simulink model "sschdlexMMCModel"  (R2026a)
settings: Solver=FixedStepDiscrete  StopTime=0.5
PostLoadFcn:
  | N = 5; % Number of Half-bridge Sub modules
  | Vdc = 640e3; % Input DC Voltage
InitFcn:
  | % Controller Parameters
  | m = 0.8; % Modulation Index of reference AC signals
  | f_out = 60; % Frequency of reference AC signals
  | Ts_CPU = 5e-5; % CPU sample time
  | 
  | % Plant Parameters
  | Ld = 30e-3; % Arm Inductance
  | Rd = 5; % Arm Resistance
  | Cm = 2e-3; % Capacitance
  | RL = 232.5; % Load Resistance
  | L = 50e-3; % Load Inductance
  | Ts_FPGA = 1e-6; % FPGA sample time
  | 
  | % PWM Generator Parameters
  | fsw = 1000; % Switching frequency
  | Tper = 1/(fsw); % Time period
  | Tdelay = 0:Tper/N:Tper*(N-1)/N; % Delay in the carrier signals
undefined symbols (not defined in the file or in its folder): DiscIntNeverNeededParam
libraries: fl_lib x30, nesl_utility x21, ee_lib x9
settings Model: DataTypeOverride=Off  Creator=The MathWorks, Inc.  LastModifiedBy=The MathWorks, Inc.
settings OptimizationCC: ConditionallyExecuteInputs=off  InheritOutputTypeSmallerThanSingle=on
settings DebuggingCC: ArtificialAlgebraicLoopMsg=error  SingleTaskRateTransMsg=error  ParameterPrecisionLossMsg=none
settings HardwareCC: ProdHWDeviceType=ASIC/FPGA->ASIC/FPGA  TargetBitPerLong=64.0  TargetBitPerPointer=64.0  TargetBitPerSizeT=64.0  TargetBitPerPtrDiffT=64.0  TargetLongLongMode=on  TargetIntDivRoundTo=Zero  TargetEndianess=LittleEndian  TargetWordSize=64.0  TargetHWDeviceType=Custom Processor->MATLAB Host Computer  ProdEqTarget=off
settings SimscapeCC: SimscapeNominalValues="[{\"value\":\"1\",\"unit\":\"A\"},{\"value\":\"1\",\"unit\":\"bar\"},{\"value\":\"1\",\"unit\":\"cm^2\"},{\"value\":\"1\",\"unit\":\"cm^3/s\"},{\"value\":\"1\",\"unit\":\"kJ/kg\"},{\"value\":\"1\",\"unit\":\"kW\"},{\"value\":\"1\",\"unit\":\"l\"},{\"value\":\"1\",\"unit\":\"N\"},{\"value\":\"1\",\"unit\":\"N*m\"},{\"value\":\"1\",\"unit\":\"V\"}]"  SimscapeLogType=none  SimscapeLogDataHistory=5000.0

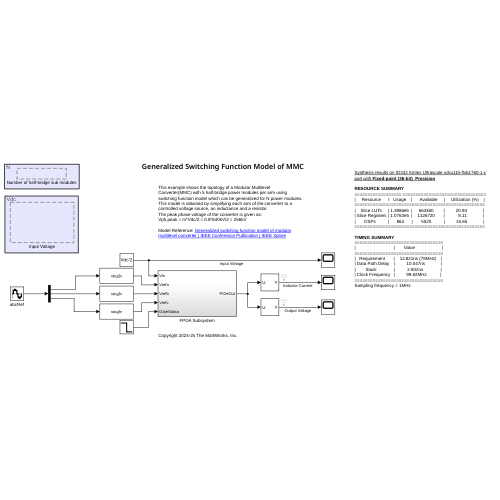
[thumbnail: Simulink's stored preview of the top-level diagram]
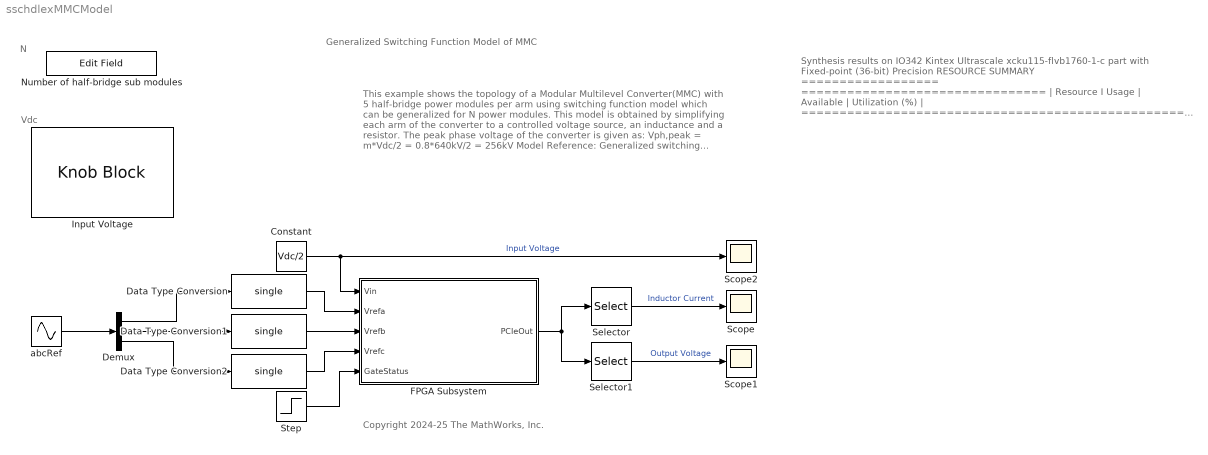
== system sschdlexMMCModel ==
  note: N
  note: Copyright 2024-25 The MathWorks, Inc.
  note: This example shows the topology of a Modular Multilevel Converter(MMC) with 5 half-bridge power modules per arm using switching function model which can be generalized for N power modules.
      | This model is obtained by simplifying each arm of the converter to a controlled voltage source, an inductance and a resistor.
      | The peak phase voltage of the converter is given as:
      | Vph,peak = m*Vdc/2 = 0.8*640kV/2 = 256kV
      |
      | Model Reference: Generalized switching function model of modular multilevel converter | IEEE Conference Publication | IEEE Xplore
  note: Synthesis results on IO342 Kintex Ultrascale xcku115-flvb1760-1-c part with Fixed-point (36-bit) Precision
      |
      | RESOURCE SUMMARY
      | ================== ================================
      | | Resource I Usage | Available | Utilization (%) |
      | ==================================================
      | | Slice LUTs | 1.3886e5 | 663360 | 20.93 |
      | | Slice Registers | 1.0763e5 | 1326720 | 8.11 |
      | | DSPs | 864 | 5520 | 15.65 |
      | ==================================================
      |
      | TIMING SUMMARY
      | ==================================
      | | | Value |
      | ==================================
      | | Requirement | 12.821ns (78MHz) |
      | | Data Path Delay | 10.047ns |
      | | Slack | 2.802ns |
      | | Clock Frequency | 99.82MHz |
      | ==================================
      | Sampling frequency = 1MHz
  note: Vdc
  note: Generalized Switching Function Model of MMC
  Constant : Constant  Value=Vdc/2  OutDataTypeStr=single  SampleTime=5e-5
  Data Type Conversion : DataTypeConversion  OutDataTypeStr=single  SaturateOnIntegerOverflow=off  RndMeth=Floor
  Data Type Conversion1 : DataTypeConversion  OutDataTypeStr=single  SaturateOnIntegerOverflow=off  RndMeth=Floor
  Data Type Conversion2 : DataTypeConversion  OutDataTypeStr=single  SaturateOnIntegerOverflow=off  RndMeth=Floor
  Demux : Demux  Outputs=3
  FPGA Subsystem : Subsystem
  Input Voltage : KnobBlock  LabelPosition=Hide  ScaleMin=2e5  ScaleMax=7e5  TickInterval=5e4
  Number of half-bridge sub modules : EditField  LabelPosition=Hide  ShowInitialText=on  Alignment=Center
  Scope : Scope
      settings: ActiveDisplayYMinimum=-1  ActiveDisplayYMaximum=1
  Scope1 : Scope
      settings: ActiveDisplayYMinimum=200918.97954337002  ActiveDisplayYMaximum=313521.80825799267  DataLoggingVariableName=ScopeData2
  Scope2 : Scope
      settings: ActiveDisplayYMinimum=220000  ActiveDisplayYMaximum=420000
  Selector : Selector  InputPortWidth=6  IndexOptions=Index vector (dialog)  Indices=[1:3]  OutputSizes=1
  Selector1 : Selector  InputPortWidth=6  IndexOptions=Index vector (dialog)  Indices=[4:6]  OutputSizes=1
  Step : Step  Time=0.25  InitialValue=1  FinalValue=0  SampleTime=5e-5
  abcRef : Sin  Amplitude=m  Frequency=2*pi*f_out  Phase=[0 -2*pi/3 2*pi/3]  SampleTime=Ts_CPU
  wires:
  Demux/1 -> Data Type Conversion/1
  Data Type Conversion1/1 -> FPGA Subsystem/3(Vrefb)
  Selector/1 -> Scope/1  "Inductor Current"
  Data Type Conversion2/1 -> FPGA Subsystem/4(Vrefc)
  Demux/3 -> Data Type Conversion2/1
  Demux/2 -> Data Type Conversion1/1
  FPGA Subsystem/1(PCIeOut) -> Selector1/1, Selector/1
  abcRef/1 -> Demux/1
  Selector1/1 -> Scope1/1  "Output Voltage"
  Constant/1 -> FPGA Subsystem/1(Vin), Scope2/1  "Input Voltage"
  Data Type Conversion/1 -> FPGA Subsystem/2(Vrefa)
  Step/1 -> FPGA Subsystem/5(GateStatus)

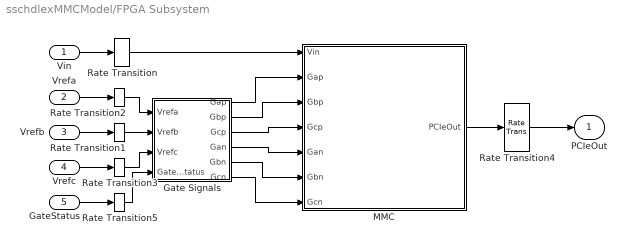
== system sschdlexMMCModel/FPGA Subsystem ==
  Vin : Inport
  Vrefa : Inport  Port=2
  Vrefb : Inport  Port=3
  Vrefc : Inport  Port=4
  GateStatus : Inport  Port=5
  Gate Signals : Subsystem
  MMC : Subsystem
  Rate Transition{,1..3,5} (5 alike) : RateTransition
  Rate Transition4 : RateTransition  OutPortSampleTime=Ts_CPU
  PCIeOut : Outport
  wires:
  Vrefc/1 -> Rate Transition3/1
  Vrefb/1 -> Rate Transition1/1
  Vrefa/1 -> Rate Transition2/1
  MMC/1(PCIeOut) -> Rate Transition4/1
  Vin/1 -> Rate Transition/1
  Rate Transition1/1 -> Gate Signals/2(Vrefb)
  Rate Transition2/1 -> Gate Signals/1(Vrefa)
  Rate Transition3/1 -> Gate Signals/3(Vrefc)
  Rate Transition4/1 -> PCIeOut/1
  Rate Transition/1 -> MMC/1(Vin)
  Gate Signals/1(Gap) -> MMC/2(Gap)
  Gate Signals/2(Gbp) -> MMC/3(Gbp)
  Gate Signals/3(Gcp) -> MMC/4(Gcp)
  Gate Signals/4(Gan) -> MMC/5(Gan)
  Gate Signals/5(Gbn) -> MMC/6(Gbn)
  Gate Signals/6(Gcn) -> MMC/7(Gcn)
  GateStatus/1 -> Rate Transition5/1
  Rate Transition5/1 -> Gate Signals/4(GateStatus)

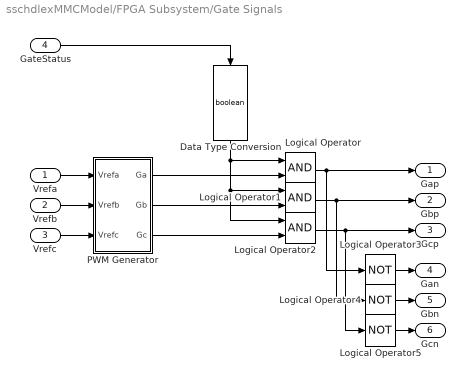
== system sschdlexMMCModel/FPGA Subsystem/Gate Signals ==
  Vrefa : Inport
  Vrefb : Inport  Port=2
  Vrefc : Inport  Port=3
  GateStatus : Inport  Port=4
  Data Type Conversion : DataTypeConversion  OutDataTypeStr=boolean  SaturateOnIntegerOverflow=off  RndMeth=Floor
  Logical Operator : Logic  AllPortsSameDT=off  OutDataTypeStr=boolean
  Logical Operator1 : Logic  AllPortsSameDT=off  OutDataTypeStr=boolean
  Logical Operator2 : Logic  AllPortsSameDT=off  OutDataTypeStr=boolean
  Logical Operator3 : Logic  Operator=NOT  AllPortsSameDT=off  OutDataTypeStr=boolean
  Logical Operator4 : Logic  Operator=NOT  AllPortsSameDT=off  OutDataTypeStr=boolean
  Logical Operator5 : Logic  Operator=NOT  AllPortsSameDT=off  OutDataTypeStr=boolean
  PWM Generator : Subsystem
  Gap : Outport
  Gbp : Outport  Port=2
  Gcp : Outport  Port=3
  Gan : Outport  Port=4
  Gbn : Outport  Port=5
  Gcn : Outport  Port=6
  wires:
  GateStatus/1 -> Data Type Conversion/1
  Logical Operator/1 -> Logical Operator3/1, Gap/1
  Data Type Conversion/1 -> Logical Operator2/1, Logical Operator1/1, Logical Operator/1
  Logical Operator2/1 -> Gcp/1, Logical Operator5/1
  Logical Operator1/1 -> Logical Operator4/1, Gbp/1
  Logical Operator3/1 -> Gan/1
  Logical Operator4/1 -> Gbn/1
  Logical Operator5/1 -> Gcn/1
  Vrefa/1 -> PWM Generator/1(Vrefa)
  Vrefb/1 -> PWM Generator/2(Vrefb)
  Vrefc/1 -> PWM Generator/3(Vrefc)
  PWM Generator/1(Ga) -> Logical Operator/2
  PWM Generator/2(Gb) -> Logical Operator1/2
  PWM Generator/3(Gc) -> Logical Operator2/2

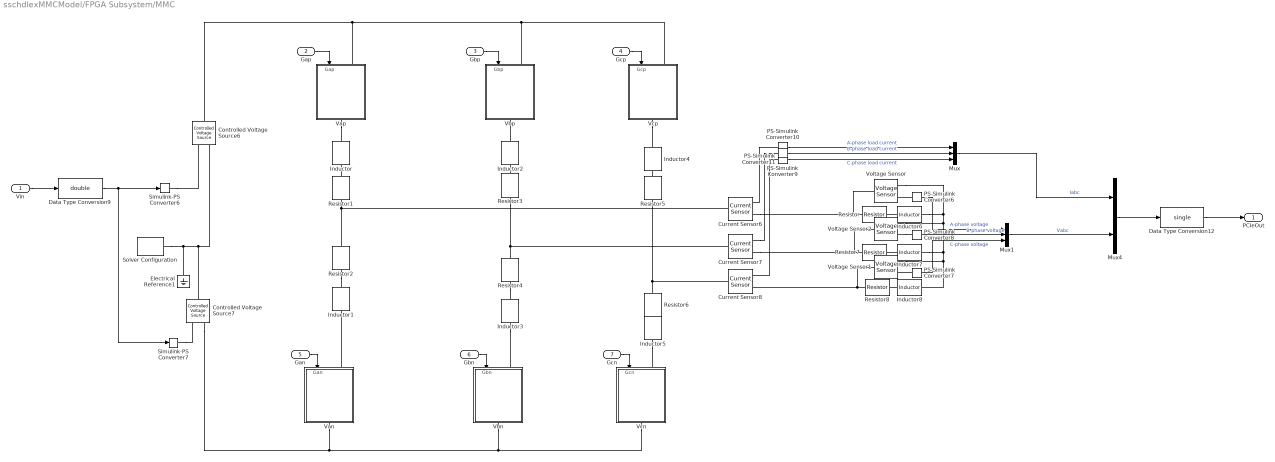
== system sschdlexMMCModel/FPGA Subsystem/MMC ==
  Vin : Inport
  Gap : Inport  Port=2
  Gbp : Inport  Port=3
  Gcp : Inport  Port=4
  Gan : Inport  Port=5
  Gbn : Inport  Port=6
  Gcn : Inport  Port=7
  Controlled Voltage Source6 : fl_lib/Electrical/Electrical Sources/Controlled Voltage Source
  Controlled Voltage Source7 : fl_lib/Electrical/Electrical Sources/Controlled Voltage Source
  Current Sensor6 : fl_lib/Electrical/Electrical Sensors/Current Sensor
  Current Sensor7 : fl_lib/Electrical/Electrical Sensors/Current Sensor
  Current Sensor8 : fl_lib/Electrical/Electrical Sensors/Current Sensor
  Data Type Conversion12 : DataTypeConversion  OutDataTypeStr=single  SaturateOnIntegerOverflow=off  RndMeth=Floor
  Data Type Conversion9 : DataTypeConversion  OutDataTypeStr=double  SaturateOnIntegerOverflow=off  RndMeth=Floor
  Electrical Reference1 : fl_lib/Electrical/Electrical Elements/Electrical Reference
  Inductor{,1..5} (6 alike) : ee_lib/Passive/Inductor  l=Ld H  enable_L_tol=ee.enum.toleranceApplication.none  L_tol=20  tol_distribution=ee.enum.toleranceDistribution.uniform  nSigma=4  r=0 Ohm  g=1e-9 1/Ohm  enable_operating_limits=ee.enum.enable.no  operating_limit_action=ee.enum.passive.reportOpLim.warn  max_working_current=1 A  power_rating=1 W  i_L_specify=off  i_L_priority=High  i_L=0 A  i_L_nominal_specify=off  i_L_nominal_value=1  i_L_nominal_unit=A
  Inductor6 : ee_lib/Passive/Inductor  l=L H  enable_L_tol=ee.enum.toleranceApplication.none  L_tol=20  tol_distribution=ee.enum.toleranceDistribution.uniform  nSigma=4  r=0 Ohm  g=1e-9 1/Ohm  enable_operating_limits=ee.enum.enable.no  operating_limit_action=ee.enum.passive.reportOpLim.warn  max_working_current=1 A  power_rating=1 W  i_L_specify=off  i_L_priority=High  i_L=0 A  i_L_nominal_specify=off  i_L_nominal_value=1  i_L_nominal_unit=A
  Inductor7 : ee_lib/Passive/Inductor  l=L H  enable_L_tol=ee.enum.toleranceApplication.none  L_tol=20  tol_distribution=ee.enum.toleranceDistribution.uniform  nSigma=4  r=0 Ohm  g=1e-9 1/Ohm  enable_operating_limits=ee.enum.enable.no  operating_limit_action=ee.enum.passive.reportOpLim.warn  max_working_current=1 A  power_rating=1 W  i_L_specify=off  i_L_priority=High  i_L=0 A  i_L_nominal_specify=off  i_L_nominal_value=1  i_L_nominal_unit=A
  Inductor8 : ee_lib/Passive/Inductor  l=L H  enable_L_tol=ee.enum.toleranceApplication.none  L_tol=20  tol_distribution=ee.enum.toleranceDistribution.uniform  nSigma=4  r=0 Ohm  g=1e-9 1/Ohm  enable_operating_limits=ee.enum.enable.no  operating_limit_action=ee.enum.passive.reportOpLim.warn  max_working_current=1 A  power_rating=1 W  i_L_specify=off  i_L_priority=High  i_L=0 A  i_L_nominal_specify=off  i_L_nominal_value=1  i_L_nominal_unit=A
  Mux : Mux  Inputs=3
  Mux1 : Mux  Inputs=3
  Mux4 : Mux  Inputs=2
  PS-Simulink Converter{6..11} (6 alike) : nesl_utility/PS-Simulink Converter  PhysicalDomain=network_engine_domain  SubClassName=ps_output  LeftPortType=input  RightPortType=output  PseudoPeriodic=off  Frequencies=[]  VectorFormat=inherit  Unit=inherit  AffineConversion=off
  Resistor : fl_lib/Electrical/Electrical Elements/Resistor  R=RL Ohm  i_specify=off  i_priority=None  i=0 A  i_nominal_specify=off  i_nominal_value=1  i_nominal_unit=A  v_specify=off  v_priority=None  v=0 V  v_nominal_specify=off  v_nominal_value=1  v_nominal_unit=V
  Resistor{1..6} (6 alike) : fl_lib/Electrical/Electrical Elements/Resistor  R=Rd Ohm  i_specify=off  i_priority=None  i=0 A  i_nominal_specify=off  i_nominal_value=1  i_nominal_unit=A  v_specify=off  v_priority=None  v=0 V  v_nominal_specify=off  v_nominal_value=1  v_nominal_unit=V
  Resistor7 : fl_lib/Electrical/Electrical Elements/Resistor  R=RL Ohm  i_specify=off  i_priority=None  i=0 A  i_nominal_specify=off  i_nominal_value=1  i_nominal_unit=A  v_specify=off  v_priority=None  v=0 V  v_nominal_specify=off  v_nominal_value=1  v_nominal_unit=V
  Resistor8 : fl_lib/Electrical/Electrical Elements/Resistor  R=RL Ohm  i_specify=off  i_priority=None  i=0 A  i_nominal_specify=off  i_nominal_value=1  i_nominal_unit=A  v_specify=off  v_priority=None  v=0 V  v_nominal_specify=off  v_nominal_value=1  v_nominal_unit=V
  Simulink-PS Converter6 : nesl_utility/Simulink-PS Converter  PhysicalDomain=network_engine_domain  SubClassName=ps_input  LeftPortType=input  RightPortType=output  PseudoPeriodic=off  Frequencies=[]  NoiseDistribution=none  NoiseParameters=[]  Unit=1  AffineConversion=off  FilteringAndDerivatives=provide  SimscapeFilterOrder=1  InputFilterTimeConstant=0.001  UdotUserProvided=0
  Simulink-PS Converter7 : nesl_utility/Simulink-PS Converter  PhysicalDomain=network_engine_domain  SubClassName=ps_input  LeftPortType=input  RightPortType=output  PseudoPeriodic=off  Frequencies=[]  NoiseDistribution=none  NoiseParameters=[]  Unit=1  AffineConversion=off  FilteringAndDerivatives=provide  SimscapeFilterOrder=1  InputFilterTimeConstant=0.001  UdotUserProvided=0
  Solver Configuration : nesl_utility/Solver Configuration  PhysicalDomain=network_engine_domain  SubClassName=solver  LeftPortType=input  RightPortType=generic  Tones=[]  Harmonics=[]  SimulateNoise=off  Profile=off  UseLocalSampling=off  EnableSwitchedLinearOptims=on  FrequencyDomain=off  UseCCode=off  RelTol=0.001  AbsTol=0.001  MinStep=1e-09  ToWorkspace=off  RevertToSquareIcSolve=off  NumHomotopyIterations=100  PhasorMode=off  PhasorModeNumHarmonics=1  ConsistencySolver=NEWTON_XTOL_AFTER_FTOL  CanonicalOrdering=UNORDERED  OptimizeIntermediates=UNOPTIMIZED  IndexReductionMethod=DerivativeReplacement  DoDC=off  ResidualTolerance=1e-09  ConsistencyTolSource=GLOBAL  ConsistencyAbsTol=0.001  ConsistencyRelTol=0.001  ConsistencyTolFactor=0.001  UseLocalSolver=on  LocalSolverChoice=NE_BACKWARD_EULER_ADVANCER  ResolveIndetEquations=off  FunctionEvalNumThread=1  LocalSolverSampleTime=Ts_FPGA  DoFixedCost=off  MaxNonlinIter=3  MaxModeIter=2  ComputeImpulses=off  ImpulseIterations=2  LinearAlgebra=auto  LinearAlgebraNumThread=0  EquationFormulation=NE_TIME_EF  DelaysMemoryBudget=1024  AutomaticFiltering=on  FilteringTimeConstant=0.001  PartitionStorageMethod=AS_NEEDED  PartitionMemoryBudget=1024  PartitionMethod=ROBUST  MultibodyUseLocalSolver=off  MultibodyLocalSolverChoice=ODE1  MultibodyLocalSolverSampleTime=0.001
  Van : Subsystem
  Vap : Subsystem
  Vbn : Subsystem
  Vbp : Subsystem
  Vcn : Subsystem
  Vcp : Subsystem
  Voltage Sensor : fl_lib/Electrical/Electrical Sensors/Voltage Sensor
  Voltage Sensor1 : fl_lib/Electrical/Electrical Sensors/Voltage Sensor
  Voltage Sensor2 : fl_lib/Electrical/Electrical Sensors/Voltage Sensor
  PCIeOut : Outport
  wires:
  Data Type Conversion12/1 -> PCIeOut/1
  Gcn/1 -> Vcn/1(Gcn)
  Gbn/1 -> Vbn/1(Gbn)
  Gcp/1 -> Vcp/1(Gcp)
  Gbp/1 -> Vbp/1(Gbp)
  Gan/1 -> Van/1(Gan)
  Gap/1 -> Vap/1(Gap)
  Data Type Conversion9/1 -> Simulink-PS Converter7/1, Simulink-PS Converter6/1
  Vin/1 -> Data Type Conversion9/1
  Mux4/1 -> Data Type Conversion12/1
  Mux1/1 -> Mux4/2  "Vabc"
  Mux/1 -> Mux4/1  "Iabc"
  PS-Simulink Converter10/1 -> Mux/1  "A-phase load current"
  PS-Simulink Converter6/1 -> Mux1/1  "A-phase voltage"
  PS-Simulink Converter8/1 -> Mux1/2  "B-phase voltage"
  PS-Simulink Converter7/1 -> Mux1/3  "C-phase voltage"
  PS-Simulink Converter11/1 -> Mux/3  "C-phase load current"
  PS-Simulink Converter9/1 -> Mux/2  "B-phase load current"
  connections:
  Inductor5/RConn1 -- Vcn/LConn1
  Inductor3/RConn1 -- Vbn/LConn1
  Current Sensor6/LConn1 -- Resistor2/LConn1 -- Resistor1/RConn1
  Vap/RConn1 -- Inductor/LConn1
  Inductor2/LConn1 -- Vbp/RConn1
  Resistor1/LConn1 -- Inductor/RConn1
  Controlled Voltage Source6/LConn1 -- Vcp/LConn1 -- Vbp/LConn1 -- Vap/LConn1
  Van/LConn1 -- Inductor1/RConn1
  Simulink-PS Converter7/RConn1 -- Controlled Voltage Source7/RConn1
  Simulink-PS Converter6/RConn1 -- Controlled Voltage Source6/RConn1
  Voltage Sensor2/RConn1 -- PS-Simulink Converter8/LConn1
  Solver Configuration/RConn1 -- Electrical Reference1/LConn1 -- Controlled Voltage Source6/RConn2 -- Controlled Voltage Source7/LConn1
  Inductor7/LConn1 -- Resistor7/RConn1
  Resistor4/RConn1 -- Inductor3/LConn1
  Vcp/RConn1 -- Inductor4/LConn1
  Inductor8/LConn1 -- Resistor8/RConn1
  PS-Simulink Converter10/LConn1 -- Current Sensor6/RConn1
  Resistor2/RConn1 -- Inductor1/LConn1
  Resistor6/RConn1 -- Inductor5/LConn1
  Resistor3/LConn1 -- Inductor2/RConn1
  Inductor6/LConn1 -- Resistor/RConn1
  PS-Simulink Converter11/LConn1 -- Current Sensor8/RConn1
  Voltage Sensor2/LConn1 -- Current Sensor7/RConn2 -- Resistor7/LConn1
  Controlled Voltage Source7/RConn2 -- Vcn/RConn1 -- Vbn/RConn1 -- Van/RConn1
  PS-Simulink Converter7/LConn1 -- Voltage Sensor1/RConn1
  Current Sensor7/RConn1 -- PS-Simulink Converter9/LConn1
  Current Sensor8/LConn1 -- Resistor5/RConn1 -- Resistor6/LConn1
  Inductor6/RConn1 -- Voltage Sensor/RConn2 -- Inductor8/RConn1 -- Voltage Sensor1/RConn2 -- Inductor7/RConn1 -- Voltage Sensor2/RConn2
  Resistor5/LConn1 -- Inductor4/RConn1
  PS-Simulink Converter6/LConn1 -- Voltage Sensor/RConn1
  Current Sensor7/LConn1 -- Resistor3/RConn1 -- Resistor4/LConn1
  Voltage Sensor1/LConn1 -- Current Sensor8/RConn2 -- Resistor8/LConn1
  Resistor/LConn1 -- Current Sensor6/RConn2 -- Voltage Sensor/LConn1

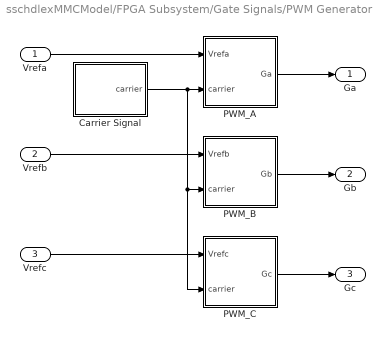
== system sschdlexMMCModel/FPGA Subsystem/Gate Signals/PWM Generator ==
  Vrefa : Inport
  Vrefb : Inport  Port=2
  Vrefc : Inport  Port=3
  Carrier Signal : Subsystem
  PWM_A : Subsystem  mask{N=N}
      mask prompts: N "Number of half-bridge sub modules"
      mask init:
      | PwmOutSelect = zeros(1,2*N);
      | PwmOutSelect(1:2:end) = 1:N;
      | PwmOutSelect(2:2:end) = N+1:2*N;
      mask DialogControl DescTextVar Prompt: PWM (a-phase)
  PWM_B : Subsystem  mask{N=N}
      mask prompts: N "Number of half-bridge sub modules"
      mask init:
      | PwmOutSelect = zeros(1,2*N);
      | PwmOutSelect(1:2:end) = 1:N;
      | PwmOutSelect(2:2:end) = N+1:2*N;
      mask DialogControl DescTextVar Prompt: PWM (b-phase)
  PWM_C : Subsystem  mask{N=N}
      mask prompts: N "Number of half-bridge sub modules"
      mask init:
      | PwmOutSelect = zeros(1,2*N);
      | PwmOutSelect(1:2:end) = 1:N;
      | PwmOutSelect(2:2:end) = N+1:2*N;
      mask DialogControl DescTextVar Prompt: PWM (c-phase)
  Ga : Outport
  Gb : Outport  Port=2
  Gc : Outport  Port=3
  wires:
  Vrefc/1 -> PWM_C/1(Vrefc)
  Vrefb/1 -> PWM_B/1(Vrefb)
  PWM_C/1(Gc) -> Gc/1
  Carrier Signal/1(carrier) -> PWM_C/2(carrier), PWM_B/2(carrier), PWM_A/2(carrier)
  Vrefa/1 -> PWM_A/1(Vrefa)
  PWM_B/1(Gb) -> Gb/1
  PWM_A/1(Ga) -> Ga/1

== system sschdlexMMCModel/FPGA Subsystem/MMC/Van ==
  Gan : Inport
  Controlled Voltage Source : fl_lib/Electrical/Electrical Sources/Controlled Voltage Source
  Current Sensor : fl_lib/Electrical/Electrical Sensors/Current Sensor
  Data Type Conversion : DataTypeConversion  OutDataTypeStr=double  SaturateOnIntegerOverflow=off  RndMeth=Floor
  Equivalent Voltage : Subsystem
  PS-Simulink Converter : nesl_utility/PS-Simulink Converter  PhysicalDomain=network_engine_domain  SubClassName=ps_output  LeftPortType=input  RightPortType=output  PseudoPeriodic=off  Frequencies=[]  VectorFormat=inherit  Unit=inherit  AffineConversion=off
  Simulink-PS Converter : nesl_utility/Simulink-PS Converter  PhysicalDomain=network_engine_domain  SubClassName=ps_input  LeftPortType=input  RightPortType=output  PseudoPeriodic=off  Frequencies=[]  NoiseDistribution=none  NoiseParameters=[]  Unit=1  AffineConversion=off  FilteringAndDerivatives=provide  SimscapeFilterOrder=1  InputFilterTimeConstant=0.001  UdotUserProvided=0
  + : PMIOPort  Side=Left
  - : PMIOPort  Port=2  Side=Right
  wires:
  Gan/1 -> Equivalent Voltage/1(Gan)
  Equivalent Voltage/1(van) -> Data Type Conversion/1
  PS-Simulink Converter/1 -> Equivalent Voltage/2(ian)
  Data Type Conversion/1 -> Simulink-PS Converter/1
  connections:
  +/RConn1 -- Controlled Voltage Source/LConn1
  Current Sensor/LConn1 -- Controlled Voltage Source/RConn2
  Current Sensor/RConn1 -- PS-Simulink Converter/LConn1
  -/RConn1 -- Current Sensor/RConn2
  Simulink-PS Converter/RConn1 -- Controlled Voltage Source/RConn1

== system sschdlexMMCModel/FPGA Subsystem/MMC/Vap ==
  Gap : Inport
  Controlled Voltage Source : fl_lib/Electrical/Electrical Sources/Controlled Voltage Source
  Current Sensor : fl_lib/Electrical/Electrical Sensors/Current Sensor
  Data Type Conversion : DataTypeConversion  OutDataTypeStr=double  SaturateOnIntegerOverflow=off  RndMeth=Floor
  Equivalent Voltage : Subsystem
  PS-Simulink Converter : nesl_utility/PS-Simulink Converter  PhysicalDomain=network_engine_domain  SubClassName=ps_output  LeftPortType=input  RightPortType=output  PseudoPeriodic=off  Frequencies=[]  VectorFormat=inherit  Unit=inherit  AffineConversion=off
  Simulink-PS Converter : nesl_utility/Simulink-PS Converter  PhysicalDomain=network_engine_domain  SubClassName=ps_input  LeftPortType=input  RightPortType=output  PseudoPeriodic=off  Frequencies=[]  NoiseDistribution=none  NoiseParameters=[]  Unit=1  AffineConversion=off  FilteringAndDerivatives=provide  SimscapeFilterOrder=1  InputFilterTimeConstant=0.001  UdotUserProvided=0
  + : PMIOPort  Side=Left
  - : PMIOPort  Port=2  Side=Right
  wires:
  Data Type Conversion/1 -> Simulink-PS Converter/1
  PS-Simulink Converter/1 -> Equivalent Voltage/2(iap)
  Equivalent Voltage/1(vap) -> Data Type Conversion/1
  Gap/1 -> Equivalent Voltage/1(Gap)
  connections:
  Simulink-PS Converter/RConn1 -- Controlled Voltage Source/RConn1
  -/RConn1 -- Current Sensor/RConn2
  Current Sensor/RConn1 -- PS-Simulink Converter/LConn1
  Current Sensor/LConn1 -- Controlled Voltage Source/RConn2
  +/RConn1 -- Controlled Voltage Source/LConn1

== system sschdlexMMCModel/FPGA Subsystem/MMC/Vbn ==
  Gbn : Inport
  Controlled Voltage Source : fl_lib/Electrical/Electrical Sources/Controlled Voltage Source
  Current Sensor : fl_lib/Electrical/Electrical Sensors/Current Sensor
  Data Type Conversion : DataTypeConversion  OutDataTypeStr=double  SaturateOnIntegerOverflow=off  RndMeth=Floor
  Equivalent Voltage : Subsystem
  PS-Simulink Converter : nesl_utility/PS-Simulink Converter  PhysicalDomain=network_engine_domain  SubClassName=ps_output  LeftPortType=input  RightPortType=output  PseudoPeriodic=off  Frequencies=[]  VectorFormat=inherit  Unit=inherit  AffineConversion=off
  Simulink-PS Converter : nesl_utility/Simulink-PS Converter  PhysicalDomain=network_engine_domain  SubClassName=ps_input  LeftPortType=input  RightPortType=output  PseudoPeriodic=off  Frequencies=[]  NoiseDistribution=none  NoiseParameters=[]  Unit=1  AffineConversion=off  FilteringAndDerivatives=provide  SimscapeFilterOrder=1  InputFilterTimeConstant=0.001  UdotUserProvided=0
  + : PMIOPort  Side=Left
  - : PMIOPort  Port=2  Side=Right
  wires:
  Data Type Conversion/1 -> Simulink-PS Converter/1
  PS-Simulink Converter/1 -> Equivalent Voltage/2(ibn)
  Equivalent Voltage/1(vbn) -> Data Type Conversion/1
  Gbn/1 -> Equivalent Voltage/1(Gbn)
  connections:
  Simulink-PS Converter/RConn1 -- Controlled Voltage Source/RConn1
  -/RConn1 -- Current Sensor/RConn2
  Current Sensor/RConn1 -- PS-Simulink Converter/LConn1
  Current Sensor/LConn1 -- Controlled Voltage Source/RConn2
  +/RConn1 -- Controlled Voltage Source/LConn1

== system sschdlexMMCModel/FPGA Subsystem/MMC/Vbp ==
  Gbp : Inport
  Controlled Voltage Source : fl_lib/Electrical/Electrical Sources/Controlled Voltage Source
  Current Sensor : fl_lib/Electrical/Electrical Sensors/Current Sensor
  Data Type Conversion : DataTypeConversion  OutDataTypeStr=double  SaturateOnIntegerOverflow=off  RndMeth=Floor
  Equivalent Voltage : Subsystem
  PS-Simulink Converter : nesl_utility/PS-Simulink Converter  PhysicalDomain=network_engine_domain  SubClassName=ps_output  LeftPortType=input  RightPortType=output  PseudoPeriodic=off  Frequencies=[]  VectorFormat=inherit  Unit=inherit  AffineConversion=off
  Simulink-PS Converter : nesl_utility/Simulink-PS Converter  PhysicalDomain=network_engine_domain  SubClassName=ps_input  LeftPortType=input  RightPortType=output  PseudoPeriodic=off  Frequencies=[]  NoiseDistribution=none  NoiseParameters=[]  Unit=1  AffineConversion=off  FilteringAndDerivatives=provide  SimscapeFilterOrder=1  InputFilterTimeConstant=0.001  UdotUserProvided=0
  + : PMIOPort  Side=Left
  - : PMIOPort  Port=2  Side=Right
  wires:
  Gbp/1 -> Equivalent Voltage/1(Gbp)
  Equivalent Voltage/1(vbp) -> Data Type Conversion/1
  PS-Simulink Converter/1 -> Equivalent Voltage/2(ibp)
  Data Type Conversion/1 -> Simulink-PS Converter/1
  connections:
  +/RConn1 -- Controlled Voltage Source/LConn1
  Current Sensor/LConn1 -- Controlled Voltage Source/RConn2
  Current Sensor/RConn1 -- PS-Simulink Converter/LConn1
  -/RConn1 -- Current Sensor/RConn2
  Simulink-PS Converter/RConn1 -- Controlled Voltage Source/RConn1

== system sschdlexMMCModel/FPGA Subsystem/MMC/Vcn ==
  Gcn : Inport
  Controlled Voltage Source : fl_lib/Electrical/Electrical Sources/Controlled Voltage Source
  Current Sensor : fl_lib/Electrical/Electrical Sensors/Current Sensor
  Data Type Conversion : DataTypeConversion  OutDataTypeStr=double  SaturateOnIntegerOverflow=off  RndMeth=Floor
  Equivalent Voltage : Subsystem
  PS-Simulink Converter : nesl_utility/PS-Simulink Converter  PhysicalDomain=network_engine_domain  SubClassName=ps_output  LeftPortType=input  RightPortType=output  PseudoPeriodic=off  Frequencies=[]  VectorFormat=inherit  Unit=inherit  AffineConversion=off
  Simulink-PS Converter : nesl_utility/Simulink-PS Converter  PhysicalDomain=network_engine_domain  SubClassName=ps_input  LeftPortType=input  RightPortType=output  PseudoPeriodic=off  Frequencies=[]  NoiseDistribution=none  NoiseParameters=[]  Unit=1  AffineConversion=off  FilteringAndDerivatives=provide  SimscapeFilterOrder=1  InputFilterTimeConstant=0.001  UdotUserProvided=0
  + : PMIOPort  Side=Left
  - : PMIOPort  Port=2  Side=Right
  wires:
  Gcn/1 -> Equivalent Voltage/1(Gcn)
  Equivalent Voltage/1(vcn) -> Data Type Conversion/1
  PS-Simulink Converter/1 -> Equivalent Voltage/2(icn)
  Data Type Conversion/1 -> Simulink-PS Converter/1
  connections:
  +/RConn1 -- Controlled Voltage Source/LConn1
  Current Sensor/LConn1 -- Controlled Voltage Source/RConn2
  Current Sensor/RConn1 -- PS-Simulink Converter/LConn1
  -/RConn1 -- Current Sensor/RConn2
  Simulink-PS Converter/RConn1 -- Controlled Voltage Source/RConn1

== system sschdlexMMCModel/FPGA Subsystem/MMC/Vcp ==
  Gcp : Inport
  Controlled Voltage Source : fl_lib/Electrical/Electrical Sources/Controlled Voltage Source
  Current Sensor : fl_lib/Electrical/Electrical Sensors/Current Sensor
  Data Type Conversion : DataTypeConversion  OutDataTypeStr=double  SaturateOnIntegerOverflow=off  RndMeth=Floor
  Equivalent Voltage : Subsystem
  PS-Simulink Converter : nesl_utility/PS-Simulink Converter  PhysicalDomain=network_engine_domain  SubClassName=ps_output  LeftPortType=input  RightPortType=output  PseudoPeriodic=off  Frequencies=[]  VectorFormat=inherit  Unit=inherit  AffineConversion=off
  Simulink-PS Converter : nesl_utility/Simulink-PS Converter  PhysicalDomain=network_engine_domain  SubClassName=ps_input  LeftPortType=input  RightPortType=output  PseudoPeriodic=off  Frequencies=[]  NoiseDistribution=none  NoiseParameters=[]  Unit=1  AffineConversion=off  FilteringAndDerivatives=provide  SimscapeFilterOrder=1  InputFilterTimeConstant=0.001  UdotUserProvided=0
  + : PMIOPort  Side=Left
  - : PMIOPort  Port=2  Side=Right
  wires:
  Data Type Conversion/1 -> Simulink-PS Converter/1
  PS-Simulink Converter/1 -> Equivalent Voltage/2(icp)
  Equivalent Voltage/1(vcp) -> Data Type Conversion/1
  Gcp/1 -> Equivalent Voltage/1(Gcp)
  connections:
  Simulink-PS Converter/RConn1 -- Controlled Voltage Source/RConn1
  -/RConn1 -- Current Sensor/RConn2
  Current Sensor/RConn1 -- PS-Simulink Converter/LConn1
  Current Sensor/LConn1 -- Controlled Voltage Source/RConn2
  +/RConn1 -- Controlled Voltage Source/LConn1

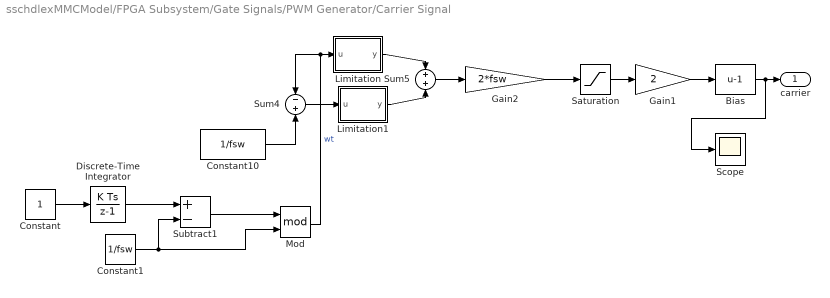
== system sschdlexMMCModel/FPGA Subsystem/Gate Signals/PWM Generator/Carrier Signal ==
  Bias : Bias  Bias=-1  SaturateOnIntegerOverflow=off
  Constant : Constant  OutDataTypeStr=single  SampleTime=-1
  Constant1 : Constant  Value=1/fsw  OutDataTypeStr=single  SampleTime=-1
  Constant10 : Constant  Value=1/fsw  OutDataTypeStr=single  SampleTime=-1
  Discrete-Time Integrator : DiscreteIntegrator  InitialCondition=Tdelay  SampleTime=-1  ICPrevOutput=DiscIntNeverNeededParam  ICPrevScaledInput=DiscIntNeverNeededParam
  Gain1 : Gain  Gain=2
  Gain2 : Gain  Gain=2*fsw
  Limitation : Subsystem
  Limitation1 : Subsystem
  Mod : Math  Operator=mod
  Saturation : Saturate  UpperLimit=1  LowerLimit=0
  Scope : Scope
      settings: ActiveDisplayYMinimum=-1.2499998658895493  ActiveDisplayYMaximum=1.2499987930059433  DataLoggingVariableName=ScopeData3
  Subtract1 : Sum  Inputs=+-
  Sum4 : Sum  Inputs=-+
  Sum5 : Sum
  carrier : Outport
  wires:
  Gain2/1 -> Saturation/1
  Saturation/1 -> Gain1/1
  Limitation/1(y) -> Sum5/1
  Subtract1/1 -> Mod/1
  Constant10/1 -> Sum4/2
  Mod/1 -> Limitation/1(u), Sum4/1  "wt"
  Constant1/1 -> Mod/2, Subtract1/2
  Sum5/1 -> Gain2/1
  Constant/1 -> Discrete-Time Integrator/1
  Gain1/1 -> Bias/1
  Limitation1/1(y) -> Sum5/2
  Discrete-Time Integrator/1 -> Subtract1/1
  Sum4/1 -> Limitation1/1(u)
  Bias/1 -> Scope/1, carrier/1

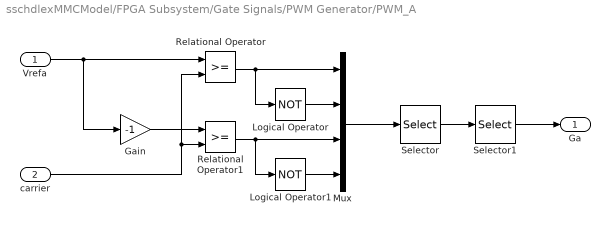
== system sschdlexMMCModel/FPGA Subsystem/Gate Signals/PWM Generator/PWM_A ==
  Vrefa : Inport
  carrier : Inport  Port=2
  Gain : Gain  Gain=-1
  Logical Operator : Logic  Operator=NOT  AllPortsSameDT=off  OutDataTypeStr=boolean
  Logical Operator1 : Logic  Operator=NOT  AllPortsSameDT=off  OutDataTypeStr=boolean
  Mux : Mux
  Relational Operator : RelationalOperator  OutDataTypeStr=boolean  RndMeth=Simplest  InputSameDT=off
  Relational Operator1 : RelationalOperator  OutDataTypeStr=boolean  RndMeth=Simplest  InputSameDT=off
  Selector : Selector  InputPortWidth=4*N  IndexOptions=Index vector (dialog)  Indices=PwmOutSelect  OutputSizes=1
  Selector1 : Selector  InputPortWidth=2*N  IndexOptions=Index vector (dialog)  Indices=[1:2:2*N]  OutputSizes=1
  Ga : Outport
  wires:
  Relational Operator1/1 -> Logical Operator1/1, Mux/3
  carrier/1 -> Relational Operator1/2, Relational Operator/2
  Vrefa/1 -> Gain/1, Relational Operator/1
  Mux/1 -> Selector/1
  Logical Operator/1 -> Mux/2
  Logical Operator1/1 -> Mux/4
  Selector/1 -> Selector1/1
  Relational Operator/1 -> Logical Operator/1, Mux/1
  Selector1/1 -> Ga/1
  Gain/1 -> Relational Operator1/1

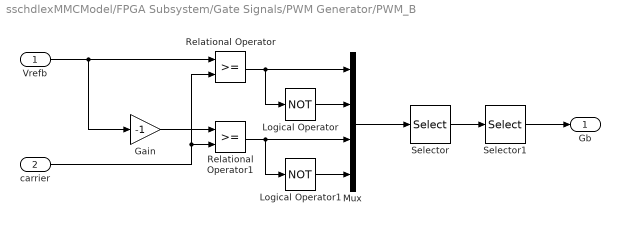
== system sschdlexMMCModel/FPGA Subsystem/Gate Signals/PWM Generator/PWM_B ==
  Vrefb : Inport
  carrier : Inport  Port=2
  Gain : Gain  Gain=-1
  Logical Operator : Logic  Operator=NOT  AllPortsSameDT=off  OutDataTypeStr=boolean
  Logical Operator1 : Logic  Operator=NOT  AllPortsSameDT=off  OutDataTypeStr=boolean
  Mux : Mux
  Relational Operator : RelationalOperator  OutDataTypeStr=boolean  RndMeth=Simplest  InputSameDT=off
  Relational Operator1 : RelationalOperator  OutDataTypeStr=boolean  RndMeth=Simplest  InputSameDT=off
  Selector : Selector  InputPortWidth=4*N  IndexOptions=Index vector (dialog)  Indices=PwmOutSelect  OutputSizes=1
  Selector1 : Selector  InputPortWidth=2*N  IndexOptions=Index vector (dialog)  Indices=[1:2:2*N]  OutputSizes=1
  Gb : Outport
  wires:
  Gain/1 -> Relational Operator1/1
  Selector1/1 -> Gb/1
  Relational Operator/1 -> Mux/1, Logical Operator/1
  Selector/1 -> Selector1/1
  Logical Operator1/1 -> Mux/4
  Logical Operator/1 -> Mux/2
  Mux/1 -> Selector/1
  Vrefb/1 -> Gain/1, Relational Operator/1
  carrier/1 -> Relational Operator/2, Relational Operator1/2
  Relational Operator1/1 -> Mux/3, Logical Operator1/1

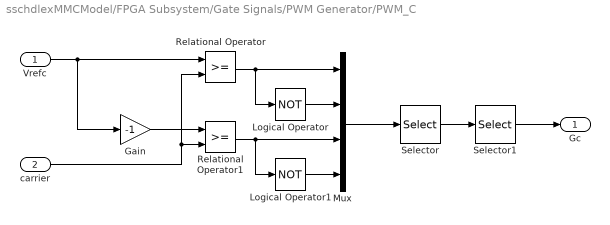
== system sschdlexMMCModel/FPGA Subsystem/Gate Signals/PWM Generator/PWM_C ==
  Vrefc : Inport
  carrier : Inport  Port=2
  Gain : Gain  Gain=-1
  Logical Operator : Logic  Operator=NOT  AllPortsSameDT=off  OutDataTypeStr=boolean
  Logical Operator1 : Logic  Operator=NOT  AllPortsSameDT=off  OutDataTypeStr=boolean
  Mux : Mux
  Relational Operator : RelationalOperator  OutDataTypeStr=boolean  RndMeth=Simplest  InputSameDT=off
  Relational Operator1 : RelationalOperator  OutDataTypeStr=boolean  RndMeth=Simplest  InputSameDT=off
  Selector : Selector  InputPortWidth=4*N  IndexOptions=Index vector (dialog)  Indices=PwmOutSelect  OutputSizes=1
  Selector1 : Selector  InputPortWidth=2*N  IndexOptions=Index vector (dialog)  Indices=[1:2:2*N]  OutputSizes=1
  Gc : Outport
  wires:
  Relational Operator1/1 -> Logical Operator1/1, Mux/3
  carrier/1 -> Relational Operator1/2, Relational Operator/2
  Vrefc/1 -> Gain/1, Relational Operator/1
  Mux/1 -> Selector/1
  Logical Operator/1 -> Mux/2
  Logical Operator1/1 -> Mux/4
  Selector/1 -> Selector1/1
  Relational Operator/1 -> Logical Operator/1, Mux/1
  Selector1/1 -> Gc/1
  Gain/1 -> Relational Operator1/1

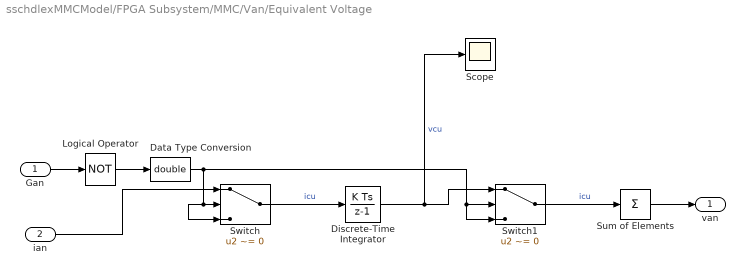
== system sschdlexMMCModel/FPGA Subsystem/MMC/Van/Equivalent Voltage ==
  Gan : Inport
  ian : Inport  Port=2
  Data Type Conversion : DataTypeConversion  OutDataTypeStr=double  SaturateOnIntegerOverflow=off  RndMeth=Floor
  Discrete-Time Integrator : DiscreteIntegrator  gainval=1/Cm  SampleTime=-1  ICPrevOutput=DiscIntNeverNeededParam  ICPrevScaledInput=DiscIntNeverNeededParam
  Logical Operator : Logic  Operator=NOT  AllPortsSameDT=off  OutDataTypeStr=boolean
  Scope : Scope
      settings: ActiveDisplayYMinimum=8640.12229  ActiveDisplayYMaximum=11210.56131  DataLoggingVariableName=ScopeData4
  Sum of Elements : Sum  Inputs=+
  Switch : Switch  Criteria=u2 ~= 0  SaturateOnIntegerOverflow=off  InputSameDT=off
  Switch1 : Switch  Criteria=u2 ~= 0  SaturateOnIntegerOverflow=off  InputSameDT=off
  van : Outport
  wires:
  Logical Operator/1 -> Data Type Conversion/1
  Switch1/1 -> Sum of Elements/1  "icu"
  ian/1 -> Switch/1
  Gan/1 -> Logical Operator/1
  Sum of Elements/1 -> van/1
  Switch/1 -> Discrete-Time Integrator/1  "icu"
  Discrete-Time Integrator/1 -> Switch1/1, Scope/1  "vcu"
  Data Type Conversion/1 -> Switch/2, Switch/3, Switch1/2, Switch1/3

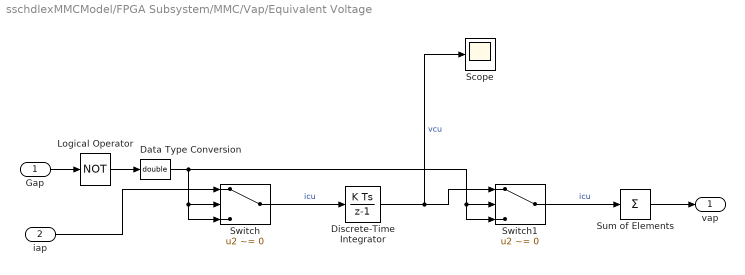
== system sschdlexMMCModel/FPGA Subsystem/MMC/Vap/Equivalent Voltage ==
  Gap : Inport
  iap : Inport  Port=2
  Data Type Conversion : DataTypeConversion  OutDataTypeStr=double  SaturateOnIntegerOverflow=off  RndMeth=Floor
  Discrete-Time Integrator : DiscreteIntegrator  gainval=1/Cm  SampleTime=-1  ICPrevOutput=DiscIntNeverNeededParam  ICPrevScaledInput=DiscIntNeverNeededParam
  Logical Operator : Logic  Operator=NOT  AllPortsSameDT=off  OutDataTypeStr=boolean
  Scope : Scope
      settings: ActiveDisplayYMinimum=8640.12229  ActiveDisplayYMaximum=11210.56131  DataLoggingVariableName=ScopeData4
  Sum of Elements : Sum  Inputs=+
  Switch : Switch  Criteria=u2 ~= 0  SaturateOnIntegerOverflow=off  InputSameDT=off
  Switch1 : Switch  Criteria=u2 ~= 0  SaturateOnIntegerOverflow=off  InputSameDT=off
  vap : Outport
  wires:
  Discrete-Time Integrator/1 -> Scope/1, Switch1/1  "vcu"
  Switch/1 -> Discrete-Time Integrator/1  "icu"
  Sum of Elements/1 -> vap/1
  Gap/1 -> Logical Operator/1
  iap/1 -> Switch/1
  Switch1/1 -> Sum of Elements/1  "icu"
  Logical Operator/1 -> Data Type Conversion/1
  Data Type Conversion/1 -> Switch1/3, Switch1/2, Switch/2, Switch/3

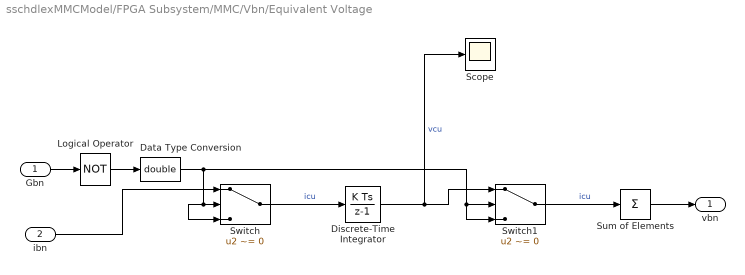
== system sschdlexMMCModel/FPGA Subsystem/MMC/Vbn/Equivalent Voltage ==
  Gbn : Inport
  ibn : Inport  Port=2
  Data Type Conversion : DataTypeConversion  OutDataTypeStr=double  SaturateOnIntegerOverflow=off  RndMeth=Floor
  Discrete-Time Integrator : DiscreteIntegrator  gainval=1/Cm  SampleTime=-1  ICPrevOutput=DiscIntNeverNeededParam  ICPrevScaledInput=DiscIntNeverNeededParam
  Logical Operator : Logic  Operator=NOT  AllPortsSameDT=off  OutDataTypeStr=boolean
  Scope : Scope
      settings: ActiveDisplayYMinimum=8640.12229  ActiveDisplayYMaximum=11210.56131  DataLoggingVariableName=ScopeData4
  Sum of Elements : Sum  Inputs=+
  Switch : Switch  Criteria=u2 ~= 0  SaturateOnIntegerOverflow=off  InputSameDT=off
  Switch1 : Switch  Criteria=u2 ~= 0  SaturateOnIntegerOverflow=off  InputSameDT=off
  vbn : Outport
  wires:
  Discrete-Time Integrator/1 -> Scope/1, Switch1/1  "vcu"
  Switch/1 -> Discrete-Time Integrator/1  "icu"
  Sum of Elements/1 -> vbn/1
  Gbn/1 -> Logical Operator/1
  ibn/1 -> Switch/1
  Switch1/1 -> Sum of Elements/1  "icu"
  Logical Operator/1 -> Data Type Conversion/1
  Data Type Conversion/1 -> Switch1/3, Switch1/2, Switch/3, Switch/2

== system sschdlexMMCModel/FPGA Subsystem/MMC/Vbp/Equivalent Voltage ==
  Gbp : Inport
  ibp : Inport  Port=2
  Data Type Conversion : DataTypeConversion  OutDataTypeStr=double  SaturateOnIntegerOverflow=off  RndMeth=Floor
  Discrete-Time Integrator : DiscreteIntegrator  gainval=1/Cm  SampleTime=-1  ICPrevOutput=DiscIntNeverNeededParam  ICPrevScaledInput=DiscIntNeverNeededParam
  Logical Operator : Logic  Operator=NOT  AllPortsSameDT=off  OutDataTypeStr=boolean
  Scope : Scope
      settings: ActiveDisplayYMinimum=8640.12229  ActiveDisplayYMaximum=11210.56131  DataLoggingVariableName=ScopeData4
  Sum of Elements : Sum  Inputs=+
  Switch : Switch  Criteria=u2 ~= 0  SaturateOnIntegerOverflow=off  InputSameDT=off
  Switch1 : Switch  Criteria=u2 ~= 0  SaturateOnIntegerOverflow=off  InputSameDT=off
  vbp : Outport
  wires:
  Logical Operator/1 -> Data Type Conversion/1
  Switch1/1 -> Sum of Elements/1  "icu"
  ibp/1 -> Switch/1
  Gbp/1 -> Logical Operator/1
  Sum of Elements/1 -> vbp/1
  Switch/1 -> Discrete-Time Integrator/1  "icu"
  Discrete-Time Integrator/1 -> Switch1/1, Scope/1  "vcu"
  Data Type Conversion/1 -> Switch/2, Switch/3, Switch1/2, Switch1/3

== system sschdlexMMCModel/FPGA Subsystem/MMC/Vcn/Equivalent Voltage ==
  Gcn : Inport
  icn : Inport  Port=2
  Data Type Conversion : DataTypeConversion  OutDataTypeStr=double  SaturateOnIntegerOverflow=off  RndMeth=Floor
  Discrete-Time Integrator : DiscreteIntegrator  gainval=1/Cm  SampleTime=-1  ICPrevOutput=DiscIntNeverNeededParam  ICPrevScaledInput=DiscIntNeverNeededParam
  Logical Operator : Logic  Operator=NOT  AllPortsSameDT=off  OutDataTypeStr=boolean
  Scope : Scope
      settings: ActiveDisplayYMinimum=8640.12229  ActiveDisplayYMaximum=11210.56131  DataLoggingVariableName=ScopeData4
  Sum of Elements : Sum  Inputs=+
  Switch : Switch  Criteria=u2 ~= 0  SaturateOnIntegerOverflow=off  InputSameDT=off
  Switch1 : Switch  Criteria=u2 ~= 0  SaturateOnIntegerOverflow=off  InputSameDT=off
  vcn : Outport
  wires:
  Logical Operator/1 -> Data Type Conversion/1
  Switch1/1 -> Sum of Elements/1  "icu"
  icn/1 -> Switch/1
  Gcn/1 -> Logical Operator/1
  Sum of Elements/1 -> vcn/1
  Switch/1 -> Discrete-Time Integrator/1  "icu"
  Discrete-Time Integrator/1 -> Switch1/1, Scope/1  "vcu"
  Data Type Conversion/1 -> Switch/2, Switch/3, Switch1/2, Switch1/3

== system sschdlexMMCModel/FPGA Subsystem/MMC/Vcp/Equivalent Voltage ==
  Gcp : Inport
  icp : Inport  Port=2
  Data Type Conversion : DataTypeConversion  OutDataTypeStr=double  SaturateOnIntegerOverflow=off  RndMeth=Floor
  Discrete-Time Integrator : DiscreteIntegrator  gainval=1/Cm  SampleTime=-1  ICPrevOutput=DiscIntNeverNeededParam  ICPrevScaledInput=DiscIntNeverNeededParam
  Logical Operator : Logic  Operator=NOT  AllPortsSameDT=off  OutDataTypeStr=boolean
  Scope : Scope
      settings: ActiveDisplayYMinimum=8640.12229  ActiveDisplayYMaximum=11210.56131  DataLoggingVariableName=ScopeData4
  Sum of Elements : Sum  Inputs=+
  Switch : Switch  Criteria=u2 ~= 0  SaturateOnIntegerOverflow=off  InputSameDT=off
  Switch1 : Switch  Criteria=u2 ~= 0  SaturateOnIntegerOverflow=off  InputSameDT=off
  vcp : Outport
  wires:
  Discrete-Time Integrator/1 -> Scope/1, Switch1/1  "vcu"
  Switch/1 -> Discrete-Time Integrator/1  "icu"
  Sum of Elements/1 -> vcp/1
  Gcp/1 -> Logical Operator/1
  icp/1 -> Switch/1
  Switch1/1 -> Sum of Elements/1  "icu"
  Logical Operator/1 -> Data Type Conversion/1
  Data Type Conversion/1 -> Switch1/3, Switch1/2, Switch/3, Switch/2

== system sschdlexMMCModel/FPGA Subsystem/Gate Signals/PWM Generator/Carrier Signal/Limitation ==
  u : Inport
  Constant2 : Constant  Value=0  OutDataTypeStr=single  SampleTime=-1
  Switch : Switch  Criteria=u2 > Threshold  Threshold=1/(2*fsw)  SaturateOnIntegerOverflow=off  InputSameDT=off
  y : Outport  VectorParamsAs1DForOutWhenUnconnected=off
  wires:
  u/1 -> Switch/3, Switch/2
  Switch/1 -> y/1
  Constant2/1 -> Switch/1

== system sschdlexMMCModel/FPGA Subsystem/Gate Signals/PWM Generator/Carrier Signal/Limitation1 ==
  u : Inport
  Constant2 : Constant  Value=0  OutDataTypeStr=single  SampleTime=-1
  Switch : Switch  Criteria=u2 > Threshold  Threshold=1/(2*fsw)  SaturateOnIntegerOverflow=off  InputSameDT=off
  y : Outport  VectorParamsAs1DForOutWhenUnconnected=off
  wires:
  u/1 -> Switch/3, Switch/2
  Switch/1 -> y/1
  Constant2/1 -> Switch/1
